simulink model "boost_frest_sps"  (R2025a)
settings: Solver=ode23tb  StartTime=0.0  StopTime=0.5  MaxStep=5e-06  RelTol=1e-05
PreLoadFcn:
  | if ~exist('BM', 'var'), boost_mrac_params; end
InitFcn:
  | if ~exist('BM', 'var'), boost_mrac_params; end
undefined symbols (not defined in the file): BM
libraries: spsSeriesRLCBranchLib x5, spsIdealSwitchLib x2, simulink x1, spsDiodeLib x1, spsMosfetLib x1, spsControlledVoltageSourceLib x1, spsCurrentMeasurementLib x1, spsVoltageMeasurementLib x1, sps_lib x1
Description:
  | Duty-to-output plant for frestimate (Section II-A of Yanarates & Zhou 2022).
settings Model: Creator=runner  LastModifiedBy=runner
settings DataIOCC: SaveOutput=off  SignalLogging=off  SaveTime=off
settings DebuggingCC: AlgebraicLoopMsg=error

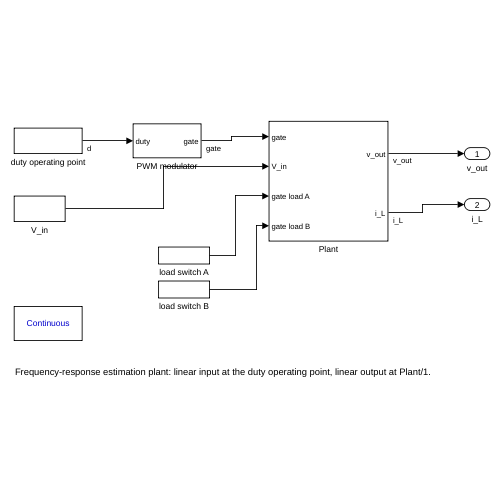
[thumbnail: Simulink's stored preview of the top-level diagram]
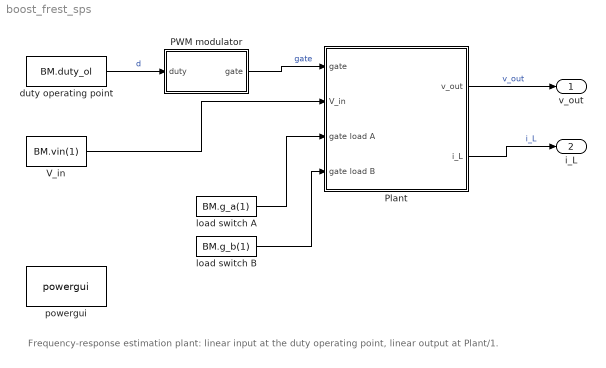
== system boost_frest_sps ==
  note: Frequency-response estimation plant: linear input at the duty operating point, linear output at Plant/1.
  PWM modulator : Subsystem
  Plant : Subsystem
  V_in : Constant  Value=BM.vin(1)
  duty operating point : Constant  Value=BM.duty_ol
  load switch A : Constant  Value=BM.g_a(1)
  load switch B : Constant  Value=BM.g_b(1)
  powergui : sps_lib/powergui  Priority=1  SimulationMode=Continuous  SampleTime=50e-6  frequency=60  Iterations=50  frequencyindice=0  Pbase=100e6  ErrMax=1e-4  UnitsV=kV  UnitsW=MW  buscounter=0  FunctionMessages=off  echomessages=off  EnableUseOfTLC=off  CurrentSourceSwitches=off  DisableSnubberDevices=off  DisableRonSwitches=off  DisableVfSwitches=off  DisplayEquations=off  AutomaticDiscreteSolvers=off  SolverType=Tustin/Backward Euler (TBE)  Interpol=off  ExternalGateDelay=off  methode=off  Ts=100  x0status=blocks  SPID=on  SwTol=0  HookPort=off  NonlinearTolerance=1e-4  nMaxIteration=100  ContinueOnMaxIteration=off  RestoreLinks=warning  ResistiveCurrentMeasurement=off  Frange=[0:2:500]  Ylog=off  Xlog=on  ShowGrid=off  save=off  variable=ZData  structure=0  ZoomFFT=off  StartTime=0.0  cycles=1  DisplayStyle=1  fundamental=60  FreqAxis=off  MaxFrequency=1000  frequencyindicesteady=1  RmsSteady=1  display=off
  v_out : Outport
  i_L : Outport  Port=2
  wires:
  duty operating point/1 -> PWM modulator/1(duty)  "d"
  load switch A/1 -> Plant/3(gate load A)
  load switch B/1 -> Plant/4(gate load B)
  PWM modulator/1(gate) -> Plant/1(gate)  "gate"
  V_in/1 -> Plant/2(V_in)
  Plant/1(v_out) -> v_out/1  "v_out"
  Plant/2(i_L) -> i_L/1  "i_L"

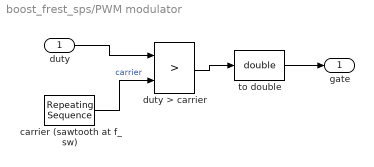
== system boost_frest_sps/PWM modulator ==
  duty : Inport
  carrier (sawtooth at f_sw) : simulink/Sources/Repeating Sequence  rep_seq_t=[0 BM.Tsw]  rep_seq_y=[0 1]
  duty > carrier : RelationalOperator  Operator=>  OutDataTypeStr=boolean  RndMeth=Simplest  InputSameDT=off
  to double : DataTypeConversion  OutDataTypeStr=double  SaturateOnIntegerOverflow=off  RndMeth=Floor
  gate : Outport
  wires:
  duty/1 -> duty > carrier/1
  carrier (sawtooth at f_sw)/1 -> duty > carrier/2  "carrier"
  duty > carrier/1 -> to double/1
  to double/1 -> gate/1

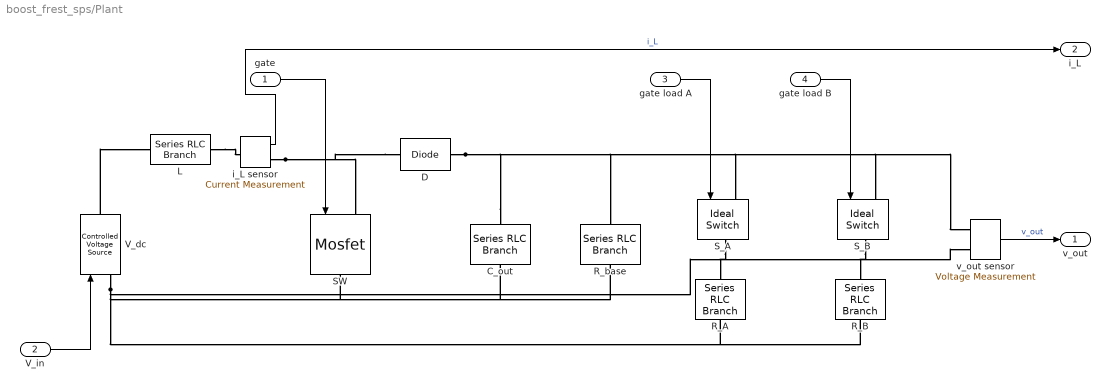
== system boost_frest_sps/Plant ==
  gate : Inport
  V_in : Inport  Port=2
  gate load A : Inport  Port=3
  gate load B : Inport  Port=4
  C_out : spsSeriesRLCBranchLib/Series RLC Branch  LConnTagsString=__new0  RConnTagsString=__new0  BranchType=C  Resistance=1  Inductance=1e-3  SetiL0=off  InitialCurrent=0  Capacitance=BM.C  Setx0=on  InitialVoltage=BM.v0  Measurements=None
  D : spsDiodeLib/Diode  Ron=BM.Ron_d  Lon=0  Vf=BM.Vf_d  IC=0  UseSnubber=0  Rs=inf  Cs=0  Measurements=off
  L : spsSeriesRLCBranchLib/Series RLC Branch  LConnTagsString=__new0  RConnTagsString=__new0  BranchType=L  Resistance=1  Inductance=BM.L  SetiL0=on  InitialCurrent=BM.iL0  Capacitance=1e-6  Setx0=off  InitialVoltage=0  Measurements=None
  R_A : spsSeriesRLCBranchLib/Series RLC Branch  LConnTagsString=__new0  RConnTagsString=__new0  BranchType=R  Resistance=BM.R_a  Inductance=1e-3  SetiL0=off  InitialCurrent=0  Capacitance=1e-6  Setx0=off  InitialVoltage=0  Measurements=None
  R_B : spsSeriesRLCBranchLib/Series RLC Branch  LConnTagsString=__new0  RConnTagsString=__new0  BranchType=R  Resistance=BM.R_b  Inductance=1e-3  SetiL0=off  InitialCurrent=0  Capacitance=1e-6  Setx0=off  InitialVoltage=0  Measurements=None
  R_base : spsSeriesRLCBranchLib/Series RLC Branch  LConnTagsString=__new0  RConnTagsString=__new0  BranchType=R  Resistance=BM.R_base  Inductance=1e-3  SetiL0=off  InitialCurrent=0  Capacitance=1e-6  Setx0=off  InitialVoltage=0  Measurements=None
  SW : spsMosfetLib/Mosfet  Ron=BM.Ron_sw  Lon=0  Rd=0.01  Vfd=0  IC=0  Rs=1e5  Cs=inf  Measurements=off
  S_A : spsIdealSwitchLib/Ideal Switch  Ron=1e-3  Lon=0  IC=0  Rs=1e5  Cs=inf  Measurements=off
  S_B : spsIdealSwitchLib/Ideal Switch  Ron=1e-3  Lon=0  IC=0  Rs=1e5  Cs=inf  Measurements=off
  V_dc : spsControlledVoltageSourceLib/Controlled Voltage Source  Initialize=on  Source_Type=DC  Amplitude=BM.vin(1)  Phase=0  Frequency=0  Measurements=None
  i_L sensor : spsCurrentMeasurementLib/Current Measurement  PhasorSimulation=off  OutputType=Complex  PSBequivalent=0
  v_out sensor : spsVoltageMeasurementLib/Voltage Measurement  PhasorSimulation=off  OutputType=Complex  PSBequivalent=0
  v_out : Outport
  i_L : Outport  Port=2
  wires:
  V_in/1 -> V_dc/1
  gate/1 -> SW/1
  gate load A/1 -> S_A/1
  gate load B/1 -> S_B/1
  i_L sensor/1 -> i_L/1  "i_L"
  v_out sensor/1 -> v_out/1  "v_out"
  connections:
  V_dc/RConn1 -- L/LConn1
  L/RConn1 -- i_L sensor/LConn1
  D/LConn1 -- i_L sensor/RConn1 -- SW/LConn1
  C_out/LConn1 -- D/RConn1 -- R_base/LConn1 -- S_A/LConn1 -- S_B/LConn1 -- v_out sensor/LConn1
  S_A/RConn1 -- R_A/LConn1
  S_B/RConn1 -- R_B/LConn1
  SW/RConn1 -- V_dc/LConn1 -- C_out/RConn1 -- R_base/RConn1 -- R_A/RConn1 -- R_B/RConn1 -- v_out sensor/LConn2
